simulink model "Lab2Sim"  (R2025b)
settings: Solver=VariableStepAuto  StartTime=0.0  StopTime=12*3600  RelTol=1e-3
values from neighbouring files (symbols this model uses):
  k = 1/580    (= 0.00172413793103)    [Lab2.m]    (also in Lab2N.m)
  P = 35960    [Lab2.m]    (also in Lab2N.m = 30740)
  Q = 937500    [Lab2.m]    (also in Lab2N.m)
  T = Q/580    (= 1616.37931034)    [Lab2.m]    (also in Lab2N.m)
settings Model: Creator=dorian  LastModifiedBy=dorian

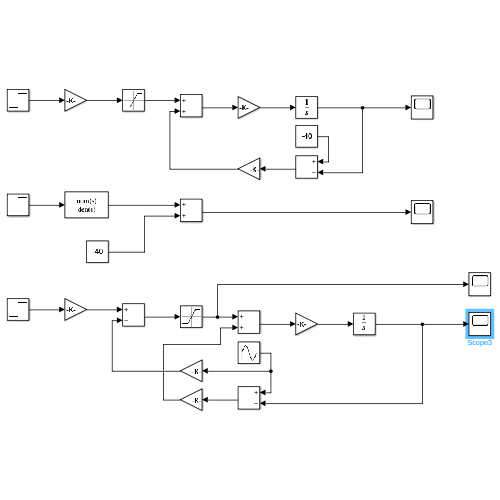
[thumbnail: Simulink's stored preview of the top-level diagram]
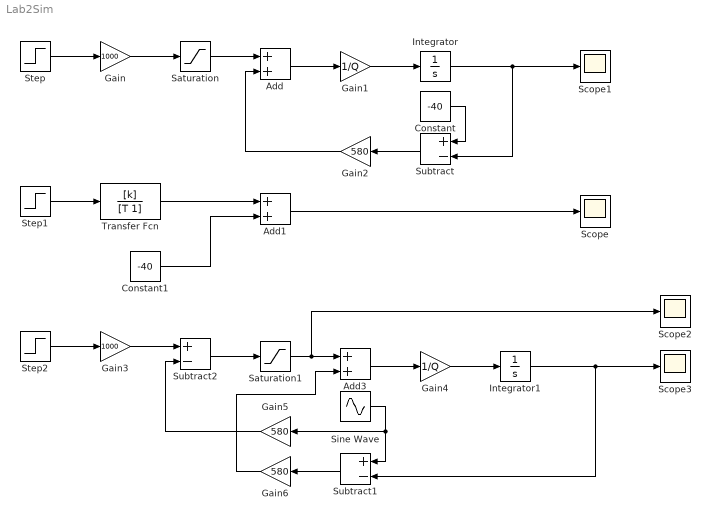
== system Lab2Sim ==
  Add : Sum
  Add1 : Sum
  Add3 : Sum
  Constant : Constant  Value=-40
  Constant1 : Constant  Value=-40
  Gain : Gain  Gain=1000
  Gain1 : Gain  Gain=1/Q
  Gain2 : Gain  Gain=580
  Gain3 : Gain  Gain=1000
  Gain4 : Gain  Gain=1/Q
  Gain5 : Gain  Gain=580
  Gain6 : Gain  Gain=580
  Integrator : Integrator
  Integrator1 : Integrator
  Saturation : Saturate  UpperLimit=P  LowerLimit=0
  Saturation1 : Saturate  UpperLimit=P  LowerLimit=0
  Scope{,1..3} (4 alike) : Scope
      Scope settings: ActiveDisplayYMinimum=-47.749987809833144  ActiveDisplayYMaximum=29.749890288498293
      Scope1 settings: ActiveDisplayYMinimum=-47.587007900594145  ActiveDisplayYMaximum=30.305313729293
      Scope2 settings: ActiveDisplayYMinimum=-1  ActiveDisplayYMaximum=1  DataLoggingVariableName=ScopeData2
      Scope3 settings: ActiveDisplayYMinimum=-8.3544864917639732  ActiveDisplayYMaximum=75.190378425875778  DataLoggingVariableName=ScopeData3
  Sine Wave : Sin  Amplitude=5  Bias=-40  Frequency=0  SampleTime=0
  Step : Step  After=24*3600  SampleTime=0
  Step1 : Step  After=P  SampleTime=0
  Step2 : Step  After=24*3600  SampleTime=0
  Subtract : Sum  Inputs=+-
  Subtract1 : Sum  Inputs=+-
  Subtract2 : Sum  Inputs=+-
  Transfer Fcn : TransferFcn  Numerator=[k]  Denominator=[T 1]
  wires:
  Step/1 -> Gain/1
  Gain/1 -> Saturation/1
  Saturation/1 -> Add/1
  Add/1 -> Gain1/1
  Gain1/1 -> Integrator/1
  Subtract/1 -> Gain2/1
  Integrator/1 -> Subtract/2, Scope1/1
  Constant/1 -> Subtract/1
  Gain2/1 -> Add/2
  Constant1/1 -> Add1/2
  Transfer Fcn/1 -> Add1/1
  Add1/1 -> Scope/1
  Step1/1 -> Transfer Fcn/1
  Step2/1 -> Gain3/1
  Gain3/1 -> Subtract2/1
  Subtract2/1 -> Saturation1/1
  Saturation1/1 -> Scope2/1, Add3/1
  Add3/1 -> Gain4/1
  Gain4/1 -> Integrator1/1
  Sine Wave/1 -> Gain5/1, Subtract1/1
  Subtract1/1 -> Gain6/1
  Gain6/1 -> Add3/2
  Gain5/1 -> Subtract2/2
  Integrator1/1 -> Subtract1/2, Scope3/1
